simulink model "DT4H_SIMULATION_EEE"  (R2025b)
settings: Solver=ode3  StartTime=0.0  StopTime=10.0  RelTol=1e-3
libraries: simulink x19, dspstat3 x6, fuzblock x1
(part 3 of 3)

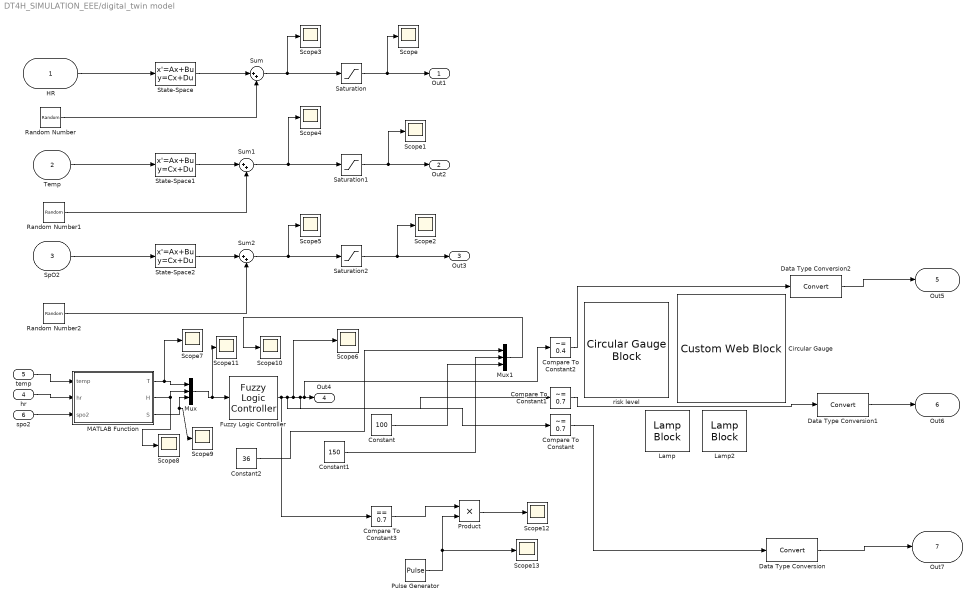
== system DT4H_SIMULATION_EEE/digital_twin model ==
  HR : Inport
  Temp : Inport  Port=2
  SpO2 : Inport  Port=3
  hr : Inport  Port=4
  temp : Inport  Port=5
  spo2 : Inport  Port=6
  Circular Gauge : CustomWebBlock  LabelPosition=Hide  ShowInitialText=on  Configuration="{\"components\":[{\"name\":\"CircularScaleComponent\",\"settings\":{\"bounds\":{\"max\":3,\"min\":0,\"tickInterval\":\"auto\"},\"direction\":\"cw\",\"flipLimits\":0,\"innerRadius\":0.75,\"internalTickHeightScaleFactor\":1,\"labelColor\":[255,255,200],\"labelFont\":{\"font\":\"Arial\",\"fontSize\":12},\"labelRadius\":0.528,\"labelTransparency\":1,\"minorTickHeightScaleFactor\":0.2,\"needleImage\":{\"size\":[200,50],\"src\":\"data:image\\/svg+xml;base64,PD94bWwgdmVyc2lvbj0iMS4wIiBlbmNvZGluZz0idXRmLTgiPz4KPCEtLSBHZW5lcmF0b3I6IEFkb2JlIElsbHVzdHJhdG9yIDI0LjEuMiwgU1ZHIEV4cG9ydCBQbHVnLUluIC4gU1ZHIFZlcnNpb246IDYuMDAgQnVpbGQgMCkgIC0tPgo8c3ZnIHZlcnNpb249IjEuMSIgaWQ9IkxheWVyXzEiIHhtbG5zPSJodHRwOi8vd3d3LnczLm9yZy8yMDAwL3N2ZyIgeG1sbnM6eGxpbms9Imh0dHA6Ly93d3cudzMub3JnLzE5OTkveGxpbmsiIHg9IjBweCIgeT0iMHB4IgoJIHZpZXdCb3g9IjAgMCAyMDAgNTAiIHN0eWxlPSJlbmFibGUtYmFja2dyb3VuZDpuZXcgMCAwIDIwMCA1MDsiIHhtbDpzcGFjZT0icHJlc2VydmUiPgo8c3R5bGUgdHlwZT0idGV4dC9jc3MiPgoJLnN0MHtmaWxsOiNFQzIxMjc7fQo8L3N0eWxlPgo8cGF0aCBjbGFzcz0ic3QwIiBkPSJNMTYyLjgsMTMuN0MxNjksNC40LDE4MS43LDEuOSwxOTEsOC4xczExLjgsMTguOSw1LjYsMjguMnMtMTguOSwxMS44LTI4LjIsNS42bDAsMAoJQzE1OS4xLDM1LjYsMTU2LjYsMjMsMTYyLjgsMTMuN0wxNjIuOCwxMy43eiBNMTY1LjgsMTUuOGMtNS4xLDcuNi0zLjEsMTcuOSw0LjYsMjNjNy42LDUuMSwxNy45LDMuMSwyMy00LjYKCWM1LjEtNy42LDMuMS0xNy45LTQuNi0yM2wwLDBDMTgxLjIsNi4yLDE3MC45LDguMiwxNjUuOCwxNS44eiIvPgo8cGF0aCBjbGFzcz0ic3QwIiBkPSJNMC40LDI1Ljl2LTMuM2wxNTktMi41Yy0wLjcsMi42LTAuNyw1LjIsMCw3LjhMMC40LDI1Ljl6Ii8+CjxjaXJjbGUgY2xhc3M9InN0MCIgY3g9IjE3OS42IiBjeT0iMjQiIHI9IjAuNyIvPgo8L3N2Zz4K\"},\"needleOffset\":[0.18464878250906522,0],\"needleOrientation\":-45,\"needleRotation\":180,\"needleSize\":{\"height\":0.11741692305346914,\"width\":0.46108337545091255},\"outerRadius\":0.9,\"position\":[0.05,0.05,0.9,0.9],\"referencePoint\":\"auto\",\"scaleAngle\":270,\"scaleAngleOffset\":135,\"scaleColors\":[],\"scaleColorsSize\":0.2,\"scaleDirection\":\"CW\",\"scalePosition\":[0,0,1,1],\"showLabels\":1,\"showMinorTicks\":1,\"showSpanLine\":1,\"showTicks\":1,\"tickColor\":[252,252,197],\"tickTransparency\":1,\"valueBarColor\":[0,114,189],\"valueBarPosition\":[0,0,1,1],\"valueBarSize\":0.2,\"valueBarTransparency\":1}},{\"name\":\"BackgroundImageComponent\",\"settings\":{\"image\":{\"size\":[500,500],\"src\":\"data:image\\/svg+xml;base64,PD94bWwgdmVyc2lvbj0iMS4wIiBlbmNvZGluZz0iVVRGLTgiIHN0YW5kYWxvbmU9Im5vIj8+CjxzdmcKICAgeG1sbnM6ZGM9Imh0dHA6Ly9wdXJsLm9yZy9kYy9lbGVtZW50cy8xLjEvIgogICB4bWxuczpjYz0iaHR0cDovL2NyZWF0aXZlY29tbW9ucy5vcmcvbnMjIgogICB4bWxuczpyZGY9Imh0dHA6Ly93d3cudzMub3JnLzE5OTkvMDIvMjItcmRmLXN5bnRheC1ucyMiCiAgIHhtbG5zOnN2Zz0iaHR0cDovL3d3dy53My5vcmcvMjAwMC9zdmciCiAgIHhtbG5zPSJodHRwOi8vd3d3LnczLm9yZy8yMDAwL3N2ZyIKICAgeG1sbnM6 ...(+9964 chars)\"},\"position\":[0,0,1,1],\"scaleMode\":\"0\"}},{\"name\":\"ForegroundImageComponent\",\"settings\":{\"image\":{\"size\":[0,0],\"src\":\"default\",\"srcOrientation\":[]},\"isForeground\":1,\"position\":[0,0,1,1],\"scaleMode\":\"0\"}}],\"derived\":{\"blockParameters\":{\"ForegroundColor\":[0.9882352941176471,0.9882352941176471,0.7725490196078432],\"Limits\":{\"Max\":3,\"Min\":0,\"Ticks\":\"auto\"},\"ScaleColors\":[],\"ScaleDirection\":\"Clockwise\",\"ScaleMax\":3,\"ScaleMin\":0,\"TickInterval\":\"auto\",\"fixedAspectRatio\":\"on\"}},\"settings\":{\"BindingType\":\"signal\",\"aspectRatio\":1.032258064516129,\"backgroundColor\":[0,0,0,\"1\"],\"backgroundOffset\":1,\"backgroundOpacity\":1,\"direction\":\"cw\",\"fixedAspectRatio\":\"on\",\"flipLimits\":0,\"orientation\":\"horizontal\",\"showBackgroundColor\":false,\"value\":0,\"version\":\"R2023a\"},\"type\":\"CircularGauge\"}"
  Compare To Constant : simulink/Logic and Bit Operations/Compare To Constant  relop=~=  const=0.7  OutDataTypeStr=boolean
  Compare To Constant1 : simulink/Logic and Bit Operations/Compare To Constant  relop=~=  const=0.7  OutDataTypeStr=boolean
  Compare To Constant2 : simulink/Logic and Bit Operations/Compare To Constant  relop=~=  const=0.4  OutDataTypeStr=boolean
  Compare To Constant3 : simulink/Logic and Bit Operations/Compare To Constant  relop===  const=0.7  OutDataTypeStr=boolean
  Constant : Constant  Value=100
  Constant1 : Constant  Value=150
  Constant2 : Constant  Value=36
  Data Type Conversion : DataTypeConversion  SaturateOnIntegerOverflow=off  RndMeth=Floor
  Data Type Conversion1 : DataTypeConversion  SaturateOnIntegerOverflow=off  RndMeth=Floor
  Data Type Conversion2 : DataTypeConversion  SaturateOnIntegerOverflow=off  RndMeth=Floor
  Fuzzy Logic Controller : fuzblock/Fuzzy Logic  Controller  FIS='HEALTH_RISK.fis'  OutputSampleNumber=101  DataType=double  UseLookupTable=off  NumBreakpoints=10  FuzzifiedInputs=off  RuleFiringStrengths=off  RuleOutputs=off  AggregatedOutputs=off  SimulateUsing=Interpreted execution  OutOfRangeInputValueMessage=warning  NoRuleFiredMessage=warning  EmptyOutputFuzzySetMessage=warning
  Lamp : LampBlock  LabelPosition=Hide  DefaultColor=[192.0, 192.0, 192.0]
  Lamp2 : LampBlock  LabelPosition=Hide  DefaultColor=[192.0, 192.0, 192.0]
  MATLAB Function : MATLAB Function  TreatAsAtomicUnit=on
  Mux : Mux  Inputs=3
  Mux1 : Mux  Inputs=3
  Product : Product
  Pulse Generator : DiscretePulseGenerator  PulseType=Time based  Period=0.1  PulseWidth=50
  Random Number : RandomNumber  Variance=0.05  SampleTime=0.01
  Random Number1 : RandomNumber  Variance=0.02  SampleTime=0.01
  Random Number2 : RandomNumber  Variance=0.01  SampleTime=0.01
  Saturation : Saturate  UpperLimit=180  LowerLimit=40
  Saturation1 : Saturate  UpperLimit=40  LowerLimit=35
  Saturation2 : Saturate  UpperLimit=100  LowerLimit=80
  Scope{,1..13} (14 alike) : Scope
      Scope settings: ActiveDisplayYMinimum=53.074255838013215  ActiveDisplayYMaximum=63.651081818656628  DataLoggingVariableName=ScopeData9  DataLoggingSaveFormat=Array
      Scope1 settings: ActiveDisplayYMinimum=24.434003490691492  ActiveDisplayYMaximum=46.484003490691492  DataLoggingVariableName=ScopeData10  DataLoggingSaveFormat=Array
      Scope10 settings: ActiveDisplayYMinimum=12.652922788173427  ActiveDisplayYMaximum=193.36816329214929  DataLoggingVariableName=ScopeData54  DataLoggingSaveFormat=Array
      Scope11 settings: ActiveDisplayYMinimum=18.641566659298462  ActiveDisplayYMaximum=57.910099346883307  DataLoggingVariableName=ScopeData55  DataLoggingSaveFormat=Array
      Scope12 settings: ActiveDisplayYMinimum=-1.3943662215757981  ActiveDisplayYMaximum=1.2858250596742027  DataLoggingVariableName=ScopeData56  DataLoggingSaveFormat=Array
      Scope13 settings: ActiveDisplayYMinimum=0.28813430571205534  ActiveDisplayYMaximum=0.6027714146457156  DataLoggingVariableName=ScopeData57  DataLoggingSaveFormat=Array
      Scope2 settings: ActiveDisplayYMinimum=68.940238419392585  ActiveDisplayYMaximum=92.092738419392589  DataLoggingVariableName=ScopeData11  DataLoggingSaveFormat=Array
      Scope3 settings: ActiveDisplayYMinimum=-0.78814818952053045  ActiveDisplayYMaximum=61.076341774502012  DataLoggingVariableName=ScopeData12  DataLoggingSaveFormat=Array
      Scope4 settings: ActiveDisplayYMinimum=-39.116379809175527  ActiveDisplayYMaximum=2.5981721305293917  DataLoggingVariableName=ScopeData13  DataLoggingSaveFormat=Array
      Scope5 settings: ActiveDisplayYMinimum=-122.44751507930864  ActiveDisplayYMaximum=30.80413037429615  DataLoggingVariableName=ScopeData14  DataLoggingSaveFormat=Array
      Scope6 settings: ActiveDisplayYMinimum=-0.43622863727232664  ActiveDisplayYMaximum=1.2187796128106578  DataLoggingVariableName=ScopeData50  DataLoggingSaveFormat=Array
      Scope7 settings: ActiveDisplayYMinimum=10.191339768848144  ActiveDisplayYMaximum=61.332204137728041  DataLoggingVariableName=ScopeData51  DataLoggingSaveFormat=Array
      Scope8 settings: ActiveDisplayYMinimum=56.268237126403491  ActiveDisplayYMaximum=63.796094453304249  DataLoggingVariableName=ScopeData52  DataLoggingSaveFormat=Array
      Scope9 settings: ActiveDisplayYMinimum=78.026041481810665  ActiveDisplayYMaximum=102.12282656778287  DataLoggingVariableName=ScopeData53  DataLoggingSaveFormat=Array
  State-Space : StateSpace  A=-1  D=0  InitialCondition=0
  State-Space1 : StateSpace  A=-0.5  B=-0.5  D=0  InitialCondition=0
  State-Space2 : StateSpace  A=-0.3  B=-0.3  D=0  InitialCondition=0
  Sum : Sum  Inputs=|++
  Sum1 : Sum  Inputs=|++
  Sum2 : Sum  Inputs=|++
  risk level : CircularGaugeBlock  ScaleMax=1  FontColor=[0.0, 0.0, 0.0]
  Out1 : Outport  VectorParamsAs1DForOutWhenUnconnected=off
  Out2 : Outport  Port=2  VectorParamsAs1DForOutWhenUnconnected=off
  Out3 : Outport  Port=3  VectorParamsAs1DForOutWhenUnconnected=off
  Out4 : Outport  Port=4
  Out5 : Outport  Port=5  VectorParamsAs1DForOutWhenUnconnected=off
  Out6 : Outport  Port=6  VectorParamsAs1DForOutWhenUnconnected=off
  Out7 : Outport  Port=7  VectorParamsAs1DForOutWhenUnconnected=off
  wires:
  HR/1 -> State-Space/1
  Temp/1 -> State-Space1/1
  SpO2/1 -> State-Space2/1
  State-Space/1 -> Sum/1
  Random Number/1 -> Sum/2
  State-Space1/1 -> Sum1/1
  Random Number1/1 -> Sum1/2
  State-Space2/1 -> Sum2/1
  Random Number2/1 -> Sum2/2
  Sum/1 -> Scope3/1, Saturation/1
  Sum1/1 -> Scope4/1, Saturation1/1
  Sum2/1 -> Scope5/1, Saturation2/1
  Saturation/1 -> Scope/1, Out1/1
  Saturation1/1 -> Scope1/1, Out2/1
  Saturation2/1 -> Scope2/1, Out3/1
  spo2/1 -> MATLAB Function/3(spo2)
  hr/1 -> MATLAB Function/2(hr)
  temp/1 -> MATLAB Function/1(temp)
  MATLAB Function/1(T) -> Scope7/1, Mux/1
  MATLAB Function/2(H) -> Scope8/1, Mux/2
  MATLAB Function/3(S) -> Scope9/1, Mux/3
  Fuzzy Logic Controller/1 -> Compare To Constant3/1, Compare To Constant/1, Scope6/1, Compare To Constant1/1, Compare To Constant2/1, Out4/1
  Constant/1 -> Mux1/3
  Constant1/1 -> Mux1/2
  Constant2/1 -> Mux1/1
  Mux1/1 -> Scope10/1
  Mux/1 -> Fuzzy Logic Controller/1, Scope11/1
  Compare To Constant/1 -> Data Type Conversion/1
  Compare To Constant1/1 -> Data Type Conversion1/1
  Compare To Constant2/1 -> Data Type Conversion2/1
  Compare To Constant3/1 -> Product/1
  Pulse Generator/1 -> Product/2, Scope13/1
  Product/1 -> Scope12/1
  Data Type Conversion2/1 -> Out5/1
  Data Type Conversion1/1 -> Out6/1
  Data Type Conversion/1 -> Out7/1

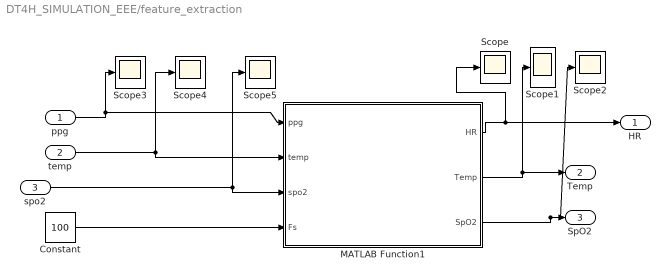
== system DT4H_SIMULATION_EEE/feature_extraction ==
  ppg : Inport
  temp : Inport  Port=2
  spo2 : Inport  Port=3
  Constant : Constant  Value=100  SampleTime=0.01
  MATLAB Function1 : MATLAB Function  TreatAsAtomicUnit=on
  Scope{,1..5} (6 alike) : Scope
      Scope settings: ActiveDisplayYMinimum=68.452333594114847  ActiveDisplayYMaximum=76.126252492955231  DataLoggingVariableName=ScopeData6  DataLoggingSaveFormat=Array
      Scope1 settings: ActiveDisplayYMinimum=34.47302672347265  ActiveDisplayYMaximum=38.552419852354959  DataLoggingVariableName=ScopeData7  DataLoggingSaveFormat=Array
      Scope2 settings: ActiveDisplayYMinimum=76.322449936569143  ActiveDisplayYMaximum=102.2491778837567  DataLoggingVariableName=ScopeData8  DataLoggingSaveFormat=Array
      Scope3 settings: ActiveDisplayYMinimum=68.2142122388407  ActiveDisplayYMaximum=80.146524249770692  DataLoggingVariableName=ScopeData62  DataLoggingSaveFormat=Array
      Scope4 settings: ActiveDisplayYMinimum=34.388543091076443  ActiveDisplayYMaximum=38.67190587640286  DataLoggingVariableName=ScopeData63  DataLoggingSaveFormat=Array
      Scope5 settings: ActiveDisplayYMinimum=76.946320036615461  ActiveDisplayYMaximum=102.873047983803  DataLoggingVariableName=ScopeData64  DataLoggingSaveFormat=Array
  HR : Outport  VectorParamsAs1DForOutWhenUnconnected=off
  Temp : Outport  Port=2  VectorParamsAs1DForOutWhenUnconnected=off
  SpO2 : Outport  Port=3  VectorParamsAs1DForOutWhenUnconnected=off
  wires:
  spo2/1 -> Scope5/1, MATLAB Function1/3(spo2)
  temp/1 -> MATLAB Function1/2(temp), Scope4/1
  ppg/1 -> Scope3/1, MATLAB Function1/1(ppg)
  Constant/1 -> MATLAB Function1/4(Fs)
  MATLAB Function1/1(HR) -> HR/1, Scope/1
  MATLAB Function1/2(Temp) -> Scope1/1, Temp/1
  MATLAB Function1/3(SpO2) -> Scope2/1, SpO2/1

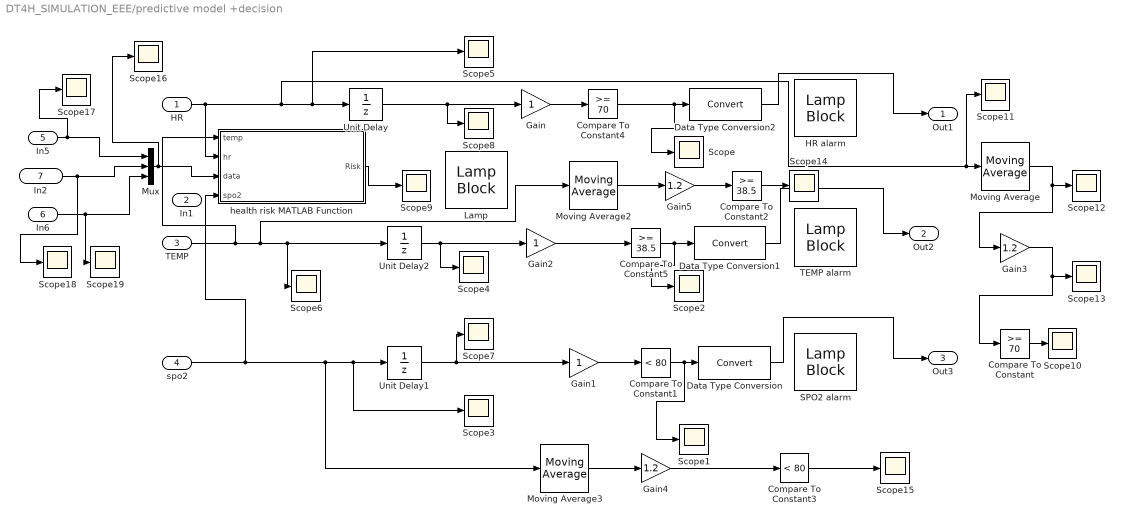
== system DT4H_SIMULATION_EEE/predictive model +decision ==
  HR : Inport
  In1 : Inport  Port=2
  TEMP : Inport  Port=3
  spo2 : Inport  Port=4
  In5 : Inport  Port=5
  In6 : Inport  Port=6
  In2 : Inport  Port=7
  Compare To Constant : simulink/Logic and Bit Operations/Compare To Constant  relop=>=  const=70  OutDataTypeStr=boolean
  Compare To Constant1 : simulink/Logic and Bit Operations/Compare To Constant  relop=<  const=80  OutDataTypeStr=boolean
  Compare To Constant2 : simulink/Logic and Bit Operations/Compare To Constant  relop=>=  const=38.5  OutDataTypeStr=boolean
  Compare To Constant3 : simulink/Logic and Bit Operations/Compare To Constant  relop=<  const=80  OutDataTypeStr=boolean
  Compare To Constant4 : simulink/Logic and Bit Operations/Compare To Constant  relop=>=  const=70  OutDataTypeStr=boolean
  Compare To Constant5 : simulink/Logic and Bit Operations/Compare To Constant  relop=>=  const=38.5  OutDataTypeStr=boolean
  Data Type Conversion : DataTypeConversion  SaturateOnIntegerOverflow=off  RndMeth=Floor
  Data Type Conversion1 : DataTypeConversion  SaturateOnIntegerOverflow=off  RndMeth=Floor
  Data Type Conversion2 : DataTypeConversion  SaturateOnIntegerOverflow=off  RndMeth=Floor
  Gain : Gain
  Gain1 : Gain
  Gain2 : Gain
  Gain3 : Gain  Gain=1.2
  Gain4 : Gain  Gain=1.2
  Gain5 : Gain  Gain=1.2
  HR alarm : LampBlock  LabelPosition=Hide  DefaultColor=[192.0, 192.0, 192.0]
  Lamp : LampBlock  LabelPosition=Hide  DefaultColor=[192.0, 192.0, 192.0]
  Moving Average : dspstat3/Moving Average  Method=Sliding window  ForgettingFactorPort=off  SpecifyWindowLength=on  WindowLength=4  OverlapLength=3  AllowArbitraryInputLength=off  ForgettingFactor=0.9  SimulateUsing=Interpreted execution
  Moving Average2 : dspstat3/Moving Average  Method=Sliding window  ForgettingFactorPort=off  SpecifyWindowLength=on  WindowLength=4  OverlapLength=3  AllowArbitraryInputLength=off  ForgettingFactor=0.9  SimulateUsing=Interpreted execution
  Moving Average3 : dspstat3/Moving Average  Method=Sliding window  ForgettingFactorPort=off  SpecifyWindowLength=on  WindowLength=4  OverlapLength=3  AllowArbitraryInputLength=off  ForgettingFactor=0.9  SimulateUsing=Interpreted execution
  Mux : Mux  Inputs=3
  SPO2 alarm : LampBlock  LabelPosition=Hide  DefaultColor=[192.0, 192.0, 192.0]
  Scope{,1..19} (20 alike) : Scope
      Scope settings: ActiveDisplayYMinimum=-0.51464394184936391  ActiveDisplayYMaximum=1.5310720166873883  DataLoggingVariableName=ScopeData15  DataLoggingSaveFormat=Array
      Scope1 settings: ActiveDisplayYMinimum=-34.596718962708131  ActiveDisplayYMaximum=23.985468310622178  DataLoggingVariableName=ScopeData16  DataLoggingSaveFormat=Array
      Scope10 settings: ActiveDisplayYMinimum=-1.1668613696808512  ActiveDisplayYMaximum=1.1483886303191491  DataLoggingVariableName=ScopeData31  DataLoggingSaveFormat=Array
      Scope11 settings: ActiveDisplayYMinimum=24.960106382978722  ActiveDisplayYMaximum=44.960106382978722  DataLoggingVariableName=ScopeData32  DataLoggingSaveFormat=Array
      Scope12 settings: ActiveDisplayYMinimum=-1  ActiveDisplayYMaximum=1  DataLoggingVariableName=ScopeData33  DataLoggingSaveFormat=Array
      Scope13 settings: ActiveDisplayYMinimum=-1  ActiveDisplayYMaximum=1  DataLoggingVariableName=ScopeData34  DataLoggingSaveFormat=Array
      Scope14 settings: ActiveDisplayYMinimum=-1  ActiveDisplayYMaximum=1  DataLoggingVariableName=ScopeData48  DataLoggingSaveFormat=Array
      Scope15 settings: ActiveDisplayYMinimum=-0.16138630319148939  ActiveDisplayYMaximum=1.2167386968085108  DataLoggingVariableName=ScopeData49  DataLoggingSaveFormat=Array
      Scope16 settings: ActiveDisplayYMinimum=-0.2142349073602936  ActiveDisplayYMaximum=1.7054674400883418  DataLoggingVariableName=ScopeData58  DataLoggingSaveFormat=Array
      Scope17 settings: ActiveDisplayYMinimum=-2.4843891866002044  ActiveDisplayYMaximum=5.4302899537328049  DataLoggingVariableName=ScopeData59  DataLoggingSaveFormat=Array
      Scope18 settings: ActiveDisplayYMinimum=0.40654912674289578  ActiveDisplayYMaximum=0.58795502243450581  DataLoggingVariableName=ScopeData60  DataLoggingSaveFormat=Array
      Scope19 settings: ActiveDisplayYMinimum=0.68932564362710647  ActiveDisplayYMaximum=1.3343456323698479  DataLoggingVariableName=ScopeData61  DataLoggingSaveFormat=Array
      Scope2 settings: ActiveDisplayYMinimum=-1.2617070966387445  ActiveDisplayYMaximum=1.290856028361256  DataLoggingVariableName=ScopeData17  DataLoggingSaveFormat=Array
      Scope3 settings: ActiveDisplayYMinimum=70.05539609392909  ActiveDisplayYMaximum=83.273832434530931  DataLoggingVariableName=ScopeData18  DataLoggingSaveFormat=Array
      Scope4 settings: ActiveDisplayYMinimum=38.814834727080509  ActiveDisplayYMaximum=97.600503046832742  DataLoggingVariableName=ScopeData19  DataLoggingSaveFormat=Array
      Scope5 settings: ActiveDisplayYMinimum=34.062103752019283  ActiveDisplayYMaximum=37.763200137745216  DataLoggingVariableName=ScopeData20  DataLoggingSaveFormat=Array
      Scope6 settings: ActiveDisplayYMinimum=36.877592350984386  ActiveDisplayYMaximum=63.675995390796629  DataLoggingVariableName=ScopeData27  DataLoggingSaveFormat=Array
      Scope7 settings: ActiveDisplayYMinimum=1.2402757459180549  ActiveDisplayYMaximum=94.856067183608459  DataLoggingVariableName=ScopeData28  DataLoggingSaveFormat=Array
      Scope8 settings: ActiveDisplayYMinimum=26.682676521779719  ActiveDisplayYMaximum=48.779399465333661  DataLoggingVariableName=ScopeData29  DataLoggingSaveFormat=Array
      Scope9 settings: ActiveDisplayYMinimum=0.12076543977224696  ActiveDisplayYMaximum=0.97178742100064641  DataLoggingVariableName=ScopeData2  DataLoggingSaveFormat=Array
  TEMP alarm : LampBlock  LabelPosition=Hide  DefaultColor=[192.0, 192.0, 192.0]
  Unit Delay : UnitDelay  InitialCondition=70  SampleTime=-1  HasFrameUpgradeWarning=on
  Unit Delay1 : UnitDelay  SampleTime=-1  HasFrameUpgradeWarning=on
  Unit Delay2 : UnitDelay  InitialCondition=37  SampleTime=-1  HasFrameUpgradeWarning=on
  health risk MATLAB Function : MATLAB Function  TreatAsAtomicUnit=on
  Out1 : Outport  VectorParamsAs1DForOutWhenUnconnected=off
  Out2 : Outport  Port=2  VectorParamsAs1DForOutWhenUnconnected=off
  Out3 : Outport  Port=3  VectorParamsAs1DForOutWhenUnconnected=off
  wires:
  HR/1 -> health risk MATLAB Function/2(hr), Scope11/1, Moving Average/1, Scope5/1, Unit Delay/1
  Unit Delay/1 -> Scope8/1, Gain/1
  Unit Delay2/1 -> Gain2/1, Scope4/1
  Unit Delay1/1 -> Gain1/1, Scope7/1
  Gain2/1 -> Compare To Constant5/1
  Gain/1 -> Compare To Constant4/1
  Compare To Constant4/1 -> Scope/1, Data Type Conversion2/1
  Compare To Constant5/1 -> Scope2/1, Data Type Conversion1/1
  Compare To Constant1/1 -> Scope1/1, Data Type Conversion/1
  TEMP/1 -> health risk MATLAB Function/1(temp), Moving Average2/1, Scope6/1, Unit Delay2/1
  spo2/1 -> health risk MATLAB Function/4(spo2), Moving Average3/1, Scope3/1, Unit Delay1/1
  Data Type Conversion2/1 -> Out1/1
  Data Type Conversion1/1 -> Out2/1
  Data Type Conversion/1 -> Out3/1
  Gain1/1 -> Compare To Constant1/1
  health risk MATLAB Function/1(Risk) -> Scope9/1
  Moving Average/1 -> Gain3/1, Scope12/1
  Gain3/1 -> Scope13/1, Compare To Constant/1
  Compare To Constant/1 -> Scope10/1
  Moving Average2/1 -> Gain5/1
  Moving Average3/1 -> Gain4/1
  Gain4/1 -> Compare To Constant3/1
  Gain5/1 -> Compare To Constant2/1
  Compare To Constant3/1 -> Scope15/1
  Compare To Constant2/1 -> Scope14/1
  In5/1 -> Scope17/1, Mux/1
  In2/1 -> Scope18/1, Mux/2
  In6/1 -> Scope19/1, Mux/3
  Mux/1 -> Scope16/1, health risk MATLAB Function/3(data)

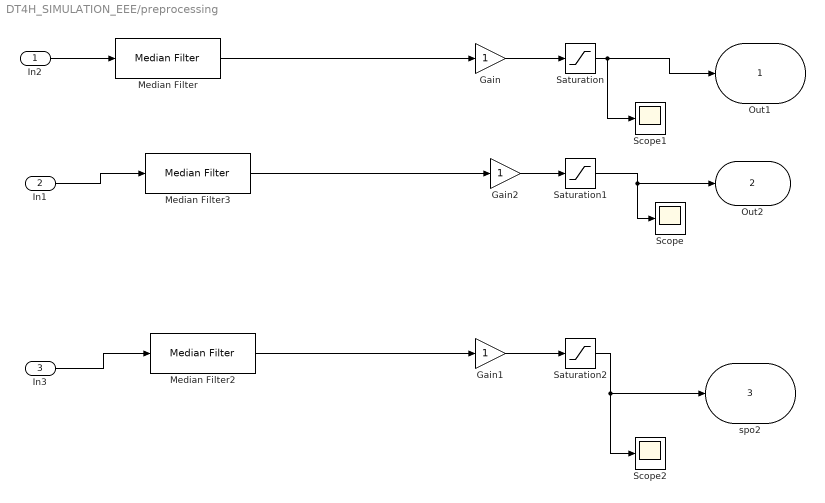
== system DT4H_SIMULATION_EEE/preprocessing ==
  In2 : Inport
  In1 : Inport  Port=2
  In3 : Inport  Port=3
  Gain : Gain
  Gain1 : Gain
  Gain2 : Gain
  Median Filter : dspstat3/Median Filter  WindowLength=7  SimulateUsing=Interpreted execution
      settings: LibrarySourceBlock=|
      | dspfdesign/Median
      | Filter
  Median Filter2 : dspstat3/Median Filter  WindowLength=10  SimulateUsing=Interpreted execution
      settings: LibrarySourceBlock=|
      | dspfdesign/Median
      | Filter
  Median Filter3 : dspstat3/Median Filter  WindowLength=15  SimulateUsing=Interpreted execution
      settings: LibrarySourceBlock=|
      | dspfdesign/Median
      | Filter
  Saturation : Saturate  UpperLimit=100  LowerLimit=60
  Saturation1 : Saturate  UpperLimit=45  LowerLimit=35
  Saturation2 : Saturate  UpperLimit=100  LowerLimit=80
  Scope : Scope
      settings: ActiveDisplayYMinimum=33.833059535887784  ActiveDisplayYMaximum=38.555467006710167  DataLoggingVariableName=ScopeData3  DataLoggingSaveFormat=Array
  Scope1 : Scope
      settings: ActiveDisplayYMinimum=34.0897954834512  ActiveDisplayYMaximum=123.88261178455774  DataLoggingVariableName=ScopeData4  DataLoggingSaveFormat=Array
  Scope2 : Scope
      settings: ActiveDisplayYMinimum=76.405769430193743  ActiveDisplayYMaximum=102.33249737738132  DataLoggingVariableName=ScopeData5  DataLoggingSaveFormat=Array
  Out1 : Outport  VectorParamsAs1DForOutWhenUnconnected=off
  Out2 : Outport  Port=2  VectorParamsAs1DForOutWhenUnconnected=off
  spo2 : Outport  Port=3  VectorParamsAs1DForOutWhenUnconnected=off
  wires:
  In1/1 -> Median Filter3/1
  In3/1 -> Median Filter2/1
  Saturation1/1 -> Scope/1, Out2/1
  Median Filter2/1 -> Gain1/1
  Saturation2/1 -> Scope2/1, spo2/1
  In2/1 -> Median Filter/1
  Median Filter/1 -> Gain/1
  Median Filter3/1 -> Gain2/1
  Gain2/1 -> Saturation1/1
  Gain1/1 -> Saturation2/1
  Gain/1 -> Saturation/1
  Saturation/1 -> Scope1/1, Out1/1

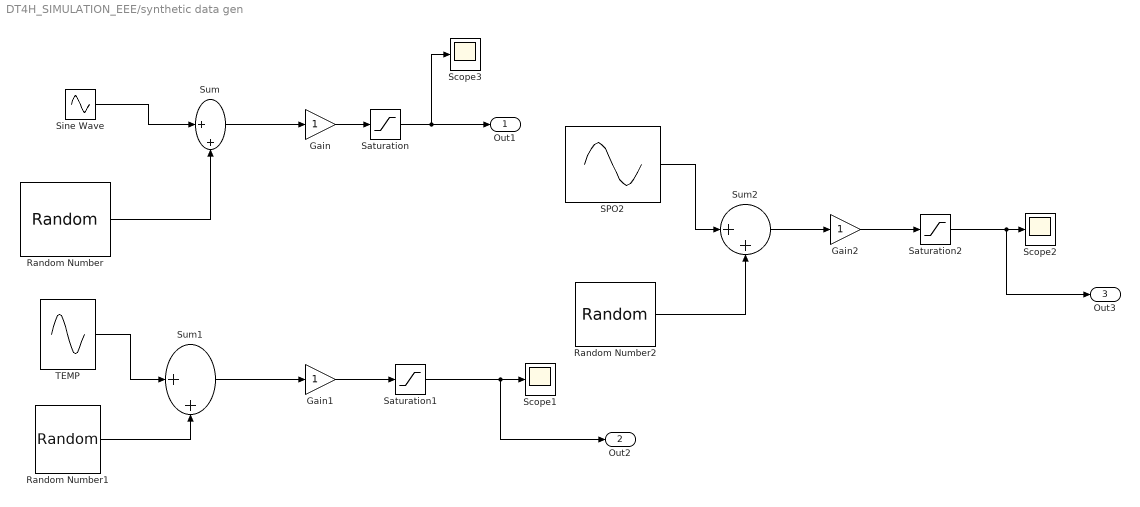
== system DT4H_SIMULATION_EEE/synthetic data gen ==
  Gain : Gain
  Gain1 : Gain
  Gain2 : Gain
  Random Number : RandomNumber  Variance=0.1  SampleTime=0.1
  Random Number1 : RandomNumber  Variance=0.05  SampleTime=0.01
  Random Number2 : RandomNumber  SampleTime=0.01
  SPO2 : Sin  Amplitude=2  Bias=97  Frequency=0.5  SampleTime=0.01
  Saturation : Saturate  UpperLimit=100  LowerLimit=80
  Saturation1 : Saturate  UpperLimit=42  LowerLimit=35
  Saturation2 : Saturate  UpperLimit=100  LowerLimit=80
  Scope1 : Scope
      settings: ActiveDisplayYMinimum=34.826479791607319  ActiveDisplayYMaximum=39.211290602772024  DataLoggingSaveFormat=Array
  Scope2 : Scope
      settings: ActiveDisplayYMinimum=94.380695326123714  ActiveDisplayYMaximum=102.51705377717757  DataLoggingSaveFormat=Array
  Scope3 : Scope
      settings: ActiveDisplayYMinimum=67.433394647606391  ActiveDisplayYMaximum=92.959025897606381  DataLoggingVariableName=ScopeData30  DataLoggingSaveFormat=Array
  Sine Wave : Sin  Frequency=7.65  SampleTime=0
  Sum : Sum  Inputs=|++
  Sum1 : Sum  Inputs=|++
  Sum2 : Sum  Inputs=|++
  TEMP : Sin  Bias=37.0  Frequency=0.5  SampleTime=0.01
  Out1 : Outport  VectorParamsAs1DForOutWhenUnconnected=off
  Out2 : Outport  Port=2  VectorParamsAs1DForOutWhenUnconnected=off
  Out3 : Outport  Port=3  VectorParamsAs1DForOutWhenUnconnected=off
  wires:
  Sine Wave/1 -> Sum/1
  Random Number/1 -> Sum/2
  Sum/1 -> Gain/1
  Random Number1/1 -> Sum1/2
  TEMP/1 -> Sum1/1
  Sum1/1 -> Gain1/1
  Gain1/1 -> Saturation1/1
  Saturation1/1 -> Out2/1, Scope1/1
  Random Number2/1 -> Sum2/2
  SPO2/1 -> Sum2/1
  Sum2/1 -> Gain2/1
  Gain2/1 -> Saturation2/1
  Saturation2/1 -> Out3/1, Scope2/1
  Gain/1 -> Saturation/1
  Saturation/1 -> Scope3/1, Out1/1

== matlab function DT4H_SIMULATION_EEE/feature_extraction/MATLAB Function1 ==
  settings: updateMethod=DISCRETE
  data: ppg input; HR output; temp input; spo2 input; Temp output; SpO2 output; Fs input
function [HR, Temp, SpO2] = extractFeatures(ppg, temp, spo2, Fs)
% Example: simple HR estimation using zero-crossings
persistent last_ppg last_time beats
if isempty(last_ppg)
    last_ppg = 0; last_time = 0; beats = 0;
end

HR = 72; 
if last_ppg < 0 && ppg >= 0
    % zero crossing detected (heartbeat)
    dt = toc;
    if dt > 0.3 && dt < 2 % valid beat interval
        HR = 60 / dt;
    end
    tic;
end
last_ppg = ppg;

% pass temperature and spo2 as-is
Temp = temp;
SpO2 = spo2;
end

== matlab function DT4H_SIMULATION_EEE/predictive model +decision/health risk MATLAB Function ==
  data: temp input; Risk output; hr input; data input; spo2 input
function Risk = Health_Risk_Index(temp, hr, data, spo2)
% Normalize inputs
t = (temp - 36) / (40 - 36);
h = (hr - 60) / (120 - 60);
s = (100 - spo2) / (100 - 80);

% Weighted combination
Risk = 0.4*t + 0.4*h + 0.2*s;

% Clamp between 0 and 1
Risk = max(0, min(1, Risk));
end

== matlab function DT4H_SIMULATION_EEE/digital_twin model/MATLAB Function ==
  data: temp input; T output; hr input; spo2 input; H output; S output
function [T, H, S] = preAdjust(temp, hr, spo2)
T = temp + randn*0.05;
H = hr + randn*1;
S = spo2 - randn*0.1;
end
